simulink model "gantry_step_count"  (R2025b)
settings: Solver=FixedStepDiscrete  StartTime=0.0  StopTime=inf  FixedStep=0.05  RelTol=1e-3  EnableMultiTasking=on
libraries: raspberrypiBasiclib x4
settings Model: Creator=jeets  LastModifiedBy=jeets
settings SolverCC: PositivePriorityOrder=on
settings OptimizationCC: EnhancedBackFolding=on  PassReuseOutputArgsAs=Individual arguments  ZeroExternalMemoryAtStartup=off  ZeroInternalMemoryAtStartup=off  MaxStackSize=200000  OptimizeBlockOrder=speed  DifferentSizesBufferReuse=on  OptimizationCustomize=off  EfficientTunableParamExpr=on
settings DebuggingCC: ParameterTunabilityLossMsg=error
settings HardwareCC: ProdBitPerPointer=32.0  ProdBitPerSizeT=32.0  ProdBitPerPtrDiffT=32.0  ProdLargestAtomicInteger=Long  ProdLargestAtomicFloat=Double  ProdWordSize=32.0  ProdLongLongMode=on  ProdHWDeviceType=ARM Compatible->ARM Cortex-A (32-bit)
settings RTWCC: SystemTargetFile=ert.tlc  HardwareBoard=Raspberry Pi  TLCOptions="-aInlineSetEventsForThisBaseRateFcn=TLC_FALSE -aSuppressMultiTaskScheduler=TLC_FALSE  -aRateBasedStepFcn=0"  TemplateMakefile=ert_default_tmf  Toolchain=GNU GCC Embedded Linux  BuildConfiguration=Faster Runs  Description=Embedded Coder
settings CodeAppCC: ForceParamTrailComments=on  IgnoreCustomStorageClasses=off  OperatorAnnotations=on  SimulinkDataObjDesc=on  SFDataObjDesc=on  InsertBlockDesc=on
settings ERTTargetCC: ExtModeTransport=2.0  ExtModeStaticAlloc=on  ExtModeMexFile=ext_xcp  ExtModeIntrfLevel=Level2 - Open  InlinedParameterPlacement=Hierarchical  CodeReplacementLibrary=ARM Cortex-A CMSIS  SupportVariableSizeSignals=on

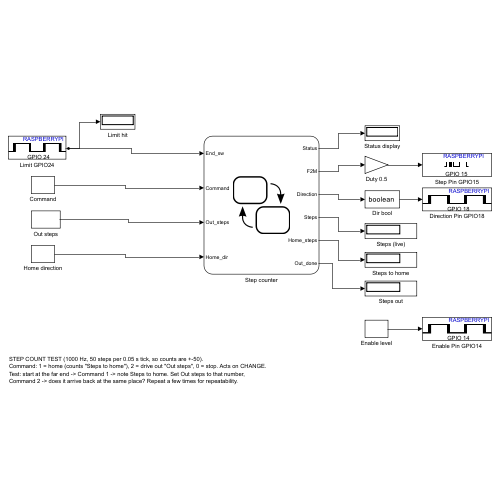
[thumbnail: Simulink's stored preview of the top-level diagram]
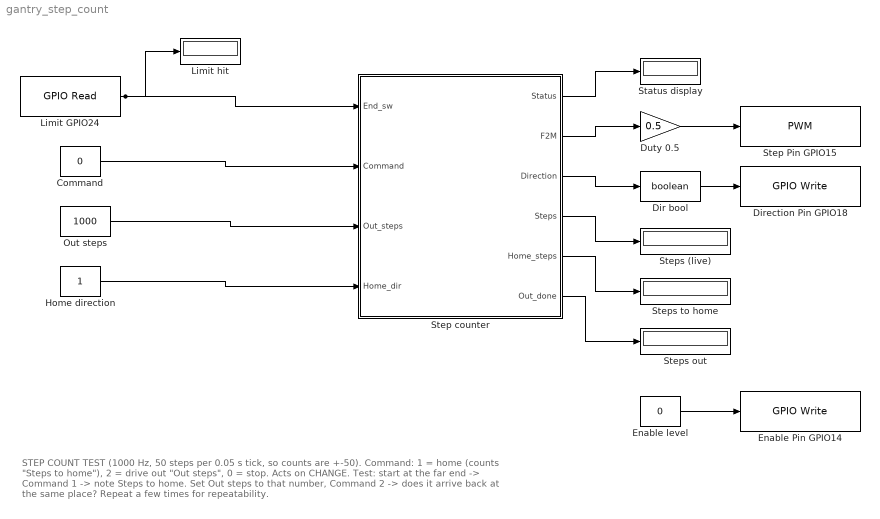
== system gantry_step_count ==
  note: STEP COUNT TEST (1000 Hz, 50 steps per 0.05 s tick, so counts are +-50).
      | Command: 1 = home (counts "Steps to home"), 2 = drive out "Out steps", 0 = stop. Acts on CHANGE.
      | Test: start at the far end -> Command 1 -> note Steps to home. Set Out steps to that number,
      | Command 2 -> does it arrive back at the same place? Repeat a few times for repeatability.
  Command : Constant  Value=0
  Dir bool : DataTypeConversion  OutDataTypeStr=boolean  SaturateOnIntegerOverflow=off  RndMeth=Floor
  Direction Pin GPIO18 : raspberrypiBasiclib/GPIO Write  BoardProperty=Pi 3 Model B+  gpio=18  blockPlatform=Raspberry Pi  PinNumber=17  board=[]  direction=[]
  Duty 0.5 : Gain  Gain=0.5
  Enable Pin GPIO14 : raspberrypiBasiclib/GPIO Write  BoardProperty=Pi 3 Model B+  gpio=14  blockPlatform=Raspberry Pi  PinNumber=17  board=[]  direction=[]
  Enable level : Constant  Value=0  OutDataTypeStr=boolean
  Home direction : Constant
  Limit GPIO24 : raspberrypiBasiclib/GPIO Read  BoardProperty=Pi 3 Model B+  gpio=24  SampleTime=0.05  blockPlatform=Raspberry Pi  PinNumber=4  board=[]  direction=[]  internalResistor=[]
  Limit hit : Display
  Out steps : Constant  Value=1000
  Status display : Display
  Step Pin GPIO15 : raspberrypiBasiclib/PWM  board=Pi 3 Model B+  Pin_=15  Frequency=1000  blockPlatform=Raspberry Pi
  Step counter : Stateflow chart  TreatAsAtomicUnit=on
  Steps (live) : Display
  Steps out : Display
  Steps to home : Display
  wires:
  Limit GPIO24/1 -> Step counter/1(End_sw), Limit hit/1
  Command/1 -> Step counter/2(Command)
  Out steps/1 -> Step counter/3(Out_steps)
  Home direction/1 -> Step counter/4(Home_dir)
  Step counter/1(Status) -> Status display/1
  Step counter/2(F2M) -> Duty 0.5/1
  Duty 0.5/1 -> Step Pin GPIO15/1
  Step counter/3(Direction) -> Dir bool/1
  Dir bool/1 -> Direction Pin GPIO18/1
  Step counter/4(Steps) -> Steps (live)/1
  Step counter/5(Home_steps) -> Steps to home/1
  Step counter/6(Out_done) -> Steps out/1
  Enable level/1 -> Enable Pin GPIO14/1

== stateflow chart gantry_step_count/Step counter ==
  settings: updateMethod=DISCRETE  sampleTime=0.05
  state Waiting
    en:
    Status = 0;
    F2M = 0;
  state Homing
    en:
    Status = 2; Steps = 0;
    Direction = Home_dir;
    F2M = 1;
    du:
    Steps = Steps + 50;
    ex:
    Steps = Steps + 50;
    Home_steps = Steps;
  state Moving_out
    en:
    Status = 3; Steps = 0; Left = 0;
    Direction = 1 - Home_dir;
    F2M = 1;
    du:
    Steps = Steps + 50;
    if End_sw == 0
    Left = 1;
    end
    ex:
    Steps = Steps + 50;
    Out_done = Steps;
  (default) -> Waiting
  Homing -> Waiting [order 1] : [End_sw == 1]
  Homing -> Waiting [order 2] : [hasChanged(Command) && Command == 0]
  Moving_out -> Waiting [order 1] : [Steps + 50 >= Out_steps]
  Moving_out -> Waiting [order 2] : [Left == 1 && End_sw == 1]
  Moving_out -> Waiting [order 3] : [hasChanged(Command) && Command == 0]
  Waiting -> Moving_out [order 2] : [hasChanged(Command) && Command == 2]
  Waiting -> Homing [order 1] : [hasChanged(Command) && Command == 1]
  data: End_sw input; Command input; Out_steps input; Home_dir input; Status output double; F2M output double; Direction output double; Steps output double; Home_steps output double; Out_done output double; Left local double =0
